simulink library "Linkage_Decoupled_Link5"  (R2025a)
settings: Solver=VariableStepAuto  StartTime=0.0  StopTime=10.0  RelTol=1e-3
undefined symbols (not defined in the file): Init, Left, Linkage, Visual, X, Y, Z
libraries: sm_lib x24, Linkage_Arms x7, Suspension_Utilities x6, Linkage_Uprights x1
(part 1 of 2)
Description:
  | Component of Simscape Vehicle Templates Library
  | 
  | Copyright 2018-2026 The MathWorks, Inc.
settings Model: Creator=smiller  LastModifiedBy=smiller
settings SolverCC: AlgebraicLoopSolver=TrustRegion
settings DataIOCC: ReturnWorkspaceOutputs=off
settings OptimizationCC: ReuseModelBlockBuffer=off
settings DebuggingCC: UnconnectedInputMsg=warning  UnconnectedOutputMsg=warning  UnconnectedLineMsg=warning  ArithmeticOperatorsInVariantConditions=warning
settings ModelReferenceCC: EnableRefExpFcnMdlSchedulingChecks=on
settings SFSimCC: CustomCodeUndefinedFunction=UseInterfaceOnly
settings RTWCC: GPUComputeCapability=3.5

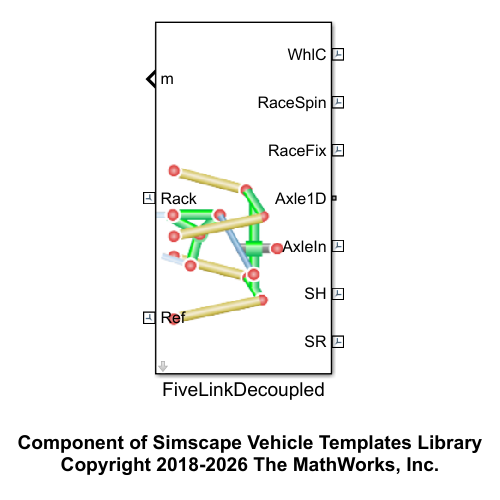
[thumbnail: Simulink's stored preview of the top-level diagram]
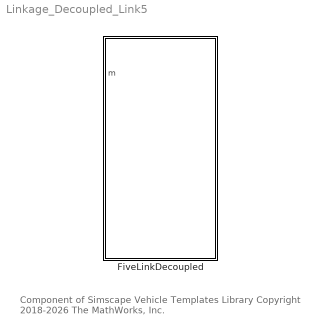
== system Linkage_Decoupled_Link5 ==
  note: Component of Simscape Vehicle Templates Library
      | Copyright 2018-2026 The MathWorks, Inc.
  FiveLinkDecoupled : Subsystem  VariantControl=FiveLinkShockFront  mask(Five-Link Suspension, Decoupled){popup_leftRight=Left, hp_in_f_ua=Linkage.UpperArmF.sInboard.Value, hp_in_r_ua=Linkage.UpperArmR.sInboard.Value, hp_out_f_ua=Linkage.UpperArmF.sOutboard.Value, hp_out_r_ua=Linkage.UpperArmR.sOutboard.Value, hp_in_f_la=Linkage.LowerArmF.sInboard.Value, hp_in_r_la=Linkage.LowerArmR.sInboard.Value, hp_out_f_la=Linkage.LowerArmF.sOutboard.Value, hp_out_r_la=Linkage.LowerArmR.sOutboard.Value, hp_pushrod_in=Linkage.Pushrod.sBellcrank.Value, hp_pushrod_out=Linkage.Pushrod.sUpright.Value, hp_bcr_pivot=Linkage.Bellcrank.sPivot.Value, hp_bcr_shock_heaveL=Linkage.Shock.sHeaveL.Value, hp_bcr_shock_heaveR=Linkage.Shock.sHeaveR.Value, hp_bcr_shock_rollL=Linkage.Shock.sRollL.Value, hp_bcr_shock_rollR=Linkage.Shock.sRollR.Value, hp_upr_cg=Linkage.Upright.sCG.Value, hp_upr_wc=Linkage.Upright.sWheelCentre.Value, hp_in_rod=Linkage.TrackRod.sInboard.Value, hp_upr_rod=Linkage.TrackRod.sOutboard.Value, clr_hp=Visual.hp.clr, opc_hp=Visual.hp.opc, size_hp=Visual.hp.rad, UpperArmF_to_Subframe=Linkage.UpperArmF_to_Subframe, UpperArmR_to_Subframe=Linkage.UpperArmR_to_Subframe, LowerArmF_to_Subframe=Linkage.LowerArmF_to_Subframe, LowerArmR_to_Subframe=Linkage.LowerArmR_to_Subframe, uaf_mass=Linkage.UpperArmF.m.Value, uar_mass=Linkage.UpperArmR.m.Value, laf_mass=Linkage.LowerArmF.m.Value, lar_mass=Linkage.LowerArmR.m.Value, clr_conn_links=Visual.hp.clr, opc_conn_links=Visual.hp.opc, size_conn_links=Visual.hp.rad, clr_uaf=Visual.UpperArm.clr, opc_uaf=Visual.part.opc, radius_uaf=Visual.UpperArm.rad, clr_uar=Visual.UpperArm.clr, opc_uar=Visual.part.opc, radius_uar=Visual.UpperArm.rad, clr_laf=Visual.LowerArm.clr, opc_laf=Visual.part.opc, radius_laf=Visual.LowerArm.rad, clr_lar=Visual.LowerArm.clr, opc_lar=Visual.part.opc, radius_lar=Visual.LowerArm.rad, atoe=Linkage.Upright.aToe.Value, acamber=Linkage.Upright.aCamber.Value, upr_mass=Linkage.Upright.m.Value, axle_len=Linkage.Upright.xAxle.Value, axle_whlc_to_bearing=Linkage.Upright.xWCtoBearing.Value, axle_mass=Linkage.Upright.mAxle.Value, clr_conn_upr=Visual.hp.clr, opc_conn_upr=Visual.hp.opc, size_conn_upr=Visual.hp.rad, clr_upr=Visual.Upright.clr, opc_upr=Visual.part.opc, radius_upr=Visual.Upright.rad, clr_axle=Visual.Axle.clr, opc_axle=Visual.part.opc, radius_axle=Visual.Axle.rad, rod_mass=Linkage.TrackRod.m.Value, clr_conn_rod=Visual.hp.clr, opc_conn_rod=Visual.hp.opc, size_conn_rod=Visual.hp.rad, clr_rod=Visual.TrackRod.clr, opc_rod=Visual.part.opc, radius_rod=Visual.TrackRod.rad, bcr_mass=Linkage.Bellcrank.m.Value, clr_bcr=Visual.Bellcrank.clr, opc_bcr=Visual.part.opc, radius_bcr=Visual.Bellcrank.rad, pushrod_mass=Linkage.Pushrod.m.Value, clr_conn_pushrod=Visual.hp.clr, opc_conn_pushrod=Visual.hp.opc, size_conn_pushrod=Visual.hp.rad, clr_pushrod=Visual.Pushrod.clr, opc_pushrod=Visual.part.opc, radius_pushrod=Visual.Pushrod.rad, whl_init_spd_lr=Init.nWheel.Value}
      mask prompts: popup_leftRight "Left/Right"; hp_in_f_ua "Upper Arm Front [xyz] (m)"; hp_in_r_ua "Upper Arm Rear [xyz] (m)"; hp_out_f_ua "Upper Arm Front Outboard [xyz] (m)"; hp_out_r_ua "Upper Arm Rear Outboard [xyz] (m)"; hp_in_f_la "Lower Arm Front [xyz] (m)"; hp_in_r_la "Lower Arm Rear [xyz] (m)"; hp_out_f_la "Lower Arm Front Outboard [xyz] (m)"; hp_out_r_la "Lower Arm Rear Outboard [xyz] (m)"; hp_pushrod_in "Pushrod Bellcrank [xyz] (m)"; hp_pushrod_out "Pushrod Upright [xyz] (m)"; hp_bcr_pivot "Bellcrank Pivot [xyz] (m)"; hp_bcr_shock_heaveL "Bellcrank Shock Heave Left [xyz] (m)"; hp_bcr_shock_heaveR "Bellcrank Shock Heave Right [xyz] (m)"; hp_bcr_shock_rollL "Bellcrank Shock Roll Left [xyz] (m)"; hp_bcr_shock_rollR "Bellcrank Shock Roll Right [xyz] (m)"; hp_upr_cg "Upright CG [xyz] (m)"; hp_upr_wc "Wheel Center [xyz] (m)"; hp_in_rod "Track Rod Inboard [xyz] (m)"; hp_upr_rod "Track Rod Outboard [xyz] (m)"; atoe "Toe Angle (deg)"; acamber "Camber Angle (deg)"; upr_mass "Mass (kg)"; axle_len "Axle Length (m)"; axle_whlc_to_bearing "Distance Wheel Ctr to Bearing (m)"; axle_mass "Axle Mass (kg)"; rod_mass "Mass (kg)"; bcr_mass "Mass (kg)"; pushrod_mass "Mass (kg)"; whl_init_spd_lr "Initial Wheel Speed (rad/s)"
      mask help: Models a multi-link, decoupled suspension with two upper and two lower control arms connecting the subframe to the upright. Mechanical connections via a bellcrank permit this design to decouple stiffness and damping for body roll and heave.
      mask init:
      | if(popup_leftRight == 1)
      |     rhs_susp = 1;
      |     %whlind = 1;
      |     whl_init_spd = whl_init_spd_lr(1);
      |     hp_bcr_shock_heave = hp_bcr_shock_heaveL;
      |     hp_bcr_shock_roll = hp_bcr_shock_rollL;
      | elseif(popup_leftRight == 2)
      |     rhs_susp = -1;
      |     %whlind = 2;
      | 	whl_init_spd = whl_init_spd_lr(2);
      |     hp_bcr_shock_heave = hp_bcr_shock_heaveR;
      |     hp_bcr_shock_roll = hp_bcr_shock_rollR;    
      | end
      mask TypeOptions popup_leftRight:
      | Hardpoints/popup_leftRight | Upright/popup_leftRight | Lower Arm Rear/popup_leftRight | Lower Arm Front/popup_leftRight | Track Rod/popup_leftRight | Upper Arm Front/popup_leftRight | Upper Arm Rear/popup_leftRight | Universal
      | HP LAF/popup_leftRight | Universal
      | HP LAR/popup_leftRight | Universal
      | HP UAF/popup_leftRight | Universal
      | HP UAR/popup_leftRight | Pushrod/popup_leftRight | Bellcrank/popup_leftRight | HP Bellcrank/popup_leftRight
      mask TypeOptions hp_in_f_ua:
      | Hardpoints/hp_in_f_ua | Universal
      | HP UAF/hp_joint | Upper Arm Front/hp_in
      mask TypeOptions hp_in_r_ua:
      | Hardpoints/hp_in_r_ua | Universal
      | HP UAR/hp_joint | Upper Arm Rear/hp_in
      mask TypeOptions hp_out_f_ua: Upper Arm Front/hp_out | Upright/hp_uaf_out
      mask TypeOptions hp_out_r_ua: Upper Arm Rear/hp_out | Upright/hp_uar_out
      mask TypeOptions hp_in_f_la:
      | Hardpoints/hp_in_f_la | Lower Arm Front/hp_in | Universal
      | HP LAF/hp_joint
      mask TypeOptions hp_in_r_la:
      | Hardpoints/hp_in_r_la | Lower Arm Rear/hp_in | Universal
      | HP LAR/hp_joint
      mask TypeOptions hp_out_f_la: Upright/hp_laf_out | Lower Arm Front/hp_out
      mask TypeOptions hp_out_r_la: Upright/hp_lar_out | Lower Arm Rear/hp_out
      mask TypeOptions hp_pushrod_in: Pushrod/hp_in | Bellcrank/hp_pushrod | HP Bellcrank/hp_pushrod_in
      mask TypeOptions hp_pushrod_out: Pushrod/hp_out | Upright/hp_pushrod
      mask TypeOptions hp_bcr_pivot: Bellcrank/hp_bcr_pivot | HP Bellcrank/hp_bcr_pivot | Hardpoints/hp_bellcrank
      mask TypeOptions hp_upr_cg: Upright/hp_upr_cg
      mask TypeOptions hp_upr_wc: Upright/hp_upr_wc
      mask TypeOptions hp_in_rod: Track Rod/hp_in
      mask TypeOptions hp_upr_rod: Track Rod/hp_out | Upright/hp_upr_rod
      mask TypeOptions clr_hp: Hardpoints/clr_hp
      mask TypeOptions opc_hp: Hardpoints/opc_hp
      mask TypeOptions size_hp: Hardpoints/size_hp
      mask TypeOptions uaf_mass: Upper Arm Front/rod_mass
      mask TypeOptions uar_mass: Upper Arm Rear/rod_mass
      mask TypeOptions laf_mass: Lower Arm Front/rod_mass
      mask TypeOptions lar_mass: Lower Arm Rear/rod_mass
      mask TypeOptions clr_conn_links: Upper Arm Front/clr_conn_rod | Upper Arm Rear/clr_conn_rod | Lower Arm Front/clr_conn_rod | Lower Arm Rear/clr_conn_rod
      mask TypeOptions opc_conn_links: Upper Arm Front/opc_conn_rod | Upper Arm Rear/opc_conn_rod | Lower Arm Front/opc_conn_rod | Lower Arm Rear/opc_conn_rod
      mask TypeOptions size_conn_links: Upper Arm Front/size_conn_rod | Upper Arm Rear/size_conn_rod | Lower Arm Front/size_conn_rod | Lower Arm Rear/size_conn_rod
      mask TypeOptions clr_uaf: Upper Arm Front/clr_rod
      mask TypeOptions opc_uaf: Upper Arm Front/opc_rod
      mask TypeOptions radius_uaf: Upper Arm Front/radius_rod
      mask TypeOptions clr_uar: Upper Arm Rear/clr_rod
      mask TypeOptions opc_uar: Upper Arm Rear/opc_rod
      mask TypeOptions radius_uar: Upper Arm Rear/radius_rod
      mask TypeOptions clr_laf: Lower Arm Front/clr_rod
      mask TypeOptions opc_laf: Lower Arm Front/opc_rod
      mask TypeOptions radius_laf: Lower Arm Front/radius_rod
      mask TypeOptions clr_lar: Lower Arm Rear/clr_rod
      mask TypeOptions opc_lar: Lower Arm Rear/opc_rod
      mask TypeOptions radius_lar: Lower Arm Rear/radius_rod
      mask TypeOptions atoe: Upright/atoe
      mask TypeOptions acamber: Upright/acamber
      mask TypeOptions upr_mass: Upright/upr_mass
      mask TypeOptions axle_len: Upright/axle_len
      mask TypeOptions axle_whlc_to_bearing: Upright/axle_whlc_to_bearing
      mask TypeOptions axle_mass: Upright/axle_mass
      mask TypeOptions clr_conn_upr: Upright/clr_conn_upr
      mask TypeOptions opc_conn_upr: Upright/opc_conn_upr
      mask TypeOptions size_conn_upr: Upright/size_conn_upr
      mask TypeOptions clr_upr: Upright/clr_upr
      mask TypeOptions opc_upr: Upright/opc_upr
      mask TypeOptions radius_upr: Upright/radius_upr
      mask TypeOptions clr_axle: Upright/clr_axle
      mask TypeOptions opc_axle: Upright/opc_axle
      mask TypeOptions radius_axle: Upright/radius_axle
      mask TypeOptions rod_mass: Track Rod/rod_mass
      mask TypeOptions clr_conn_rod: Track Rod/clr_conn_rod
      mask TypeOptions opc_conn_rod: Track Rod/opc_conn_rod
      mask TypeOptions size_conn_rod: Track Rod/size_conn_rod
      mask TypeOptions clr_rod: Track Rod/clr_rod
      mask TypeOptions opc_rod: Track Rod/opc_rod
      mask TypeOptions radius_rod: Track Rod/radius_rod
      mask TypeOptions bcr_mass: Bellcrank/bcr_mass
      mask TypeOptions clr_bcr: Bellcrank/clr_bcr
      mask TypeOptions opc_bcr: Bellcrank/opc_bcr
      mask TypeOptions radius_bcr: Bellcrank/radius_bcr
      mask TypeOptions pushrod_mass: Pushrod/rod_mass
      mask TypeOptions clr_conn_pushrod: Pushrod/clr_conn_rod
      mask TypeOptions opc_conn_pushrod: Pushrod/opc_conn_rod
      mask TypeOptions size_conn_pushrod: Pushrod/size_conn_rod
      mask TypeOptions clr_pushrod: Pushrod/clr_rod
      mask TypeOptions opc_pushrod: Pushrod/opc_rod
      mask TypeOptions radius_pushrod: Pushrod/radius_rod
      mask DialogControl cont_hp Prompt: Hardpoints
      mask DialogControl cont_vis_hp Prompt: Visualization
      mask DialogControl text_clr_hp Prompt: Color [RGB]
      mask DialogControl text_opc_hp Prompt: Opac. (0-1)
      mask DialogControl text_size_hp Prompt: Size (m)
      mask DialogControl text_hp Prompt: Hardpoints
      mask DialogControl cont_links Prompt: Links
      mask DialogControl text_links_part_subf Prompt: Part
      mask DialogControl text_links_subf Prompt: Subframe Connection
      mask DialogControl text_upper_f_subf Prompt: Upper, Front
      mask DialogControl text_upper_r_subf Prompt: Upper, Rear
      mask DialogControl text_lower_f_subf Prompt: Lower, Front
      mask DialogControl text_lower_r_subf Prompt: Lower, Rear
      mask DialogControl text_links_part Prompt: Part
      mask DialogControl text_links_mass Prompt: Mass (kg)
      mask DialogControl text_upper_f Prompt: Upper, Front
      mask DialogControl text_upper_r Prompt: Upper, Rear
      mask DialogControl text_lower_f Prompt: Lower, Front
      mask DialogControl text_lower_r Prompt: Lower, Rear
      mask DialogControl cont_vis_links Prompt: Visualization
      mask DialogControl text_vis_links_clr Prompt: Color [RGB]
      mask DialogControl text_vis_links_opc Prompt: Opacity (0-1)
      mask DialogControl text_vis_links_rad Prompt: Radius (m)
      mask DialogControl text_vis_links_conn Prompt: Connections
      mask DialogControl text_vis_links_uaf Prompt: Upper, Front
      mask DialogControl text_vis_links_uar Prompt: Upper, Rear
      mask DialogControl text_vis_links_laf Prompt: Lower, Front
      mask DialogControl text_vis_links_lar Prompt: Lower, Rear
      mask DialogControl cont_upright Prompt: Upright
      mask DialogControl grp_upright Prompt: Upright
      mask DialogControl grp_upright_axle Prompt: Axle
      mask DialogControl cont_vis_upr Prompt: Visualization
      mask DialogControl text_clr_upr Prompt: Color [RGB]
      mask DialogControl text_opc_upr Prompt: Opac. (0-1)
      mask DialogControl text_size_upr Prompt: Size (m)
      mask DialogControl text_conn_upr Prompt: Connections
      mask DialogControl text_upright Prompt: Upright
      mask DialogControl text_axle Prompt: Axle
      mask DialogControl cont_steer Prompt: Steer
      mask DialogControl grp_rod Prompt: Rod
      mask DialogControl cont_vis_rod Prompt: Visualization
      mask DialogControl text_clr_rod Prompt: Color [RGB]
      mask DialogControl text_opc_rod Prompt: Opac. (0-1)
      mask DialogControl text_size_rod Prompt: Size (m)
      mask DialogControl text_conn_rod Prompt: Connections
      mask DialogControl text_rod_rod Prompt: Rod
      mask DialogControl cont_bellcrank Prompt: Bellcrank
      mask DialogControl grp_bellcrank Prompt: Bellcrank
      mask DialogControl cont_vis_bellcrank Prompt: Visualization
      mask DialogControl text_clr_bellcrank Prompt: Color [RGB]
      mask DialogControl text_opc_bellcrank Prompt: Opac. (0-1)
      mask DialogControl text_size_bellcrank Prompt: Size (m)
      mask DialogControl text_bellcrank Prompt: Bellcrank
      mask DialogControl cont_push Prompt: Pushrod
      mask DialogControl grp_pushrod Prompt: Pushrod
      mask DialogControl cont_vis_pushrod Prompt: Visualization
      mask DialogControl text_clr_pushrod Prompt: Color [RGB]
      mask DialogControl text_opc_pushrod Prompt: Opac. (0-1)
      mask DialogControl text_size_pushrod Prompt: Size (m)
      mask DialogControl text_conn_pushrod Prompt: Connections
      mask DialogControl text_pushrod Prompt: Pushrod
      mask DialogControl cont_initial Prompt: Initial
      mask Display: image('sm_car_vehicle_linkage_5ldec_IMAGE.png');

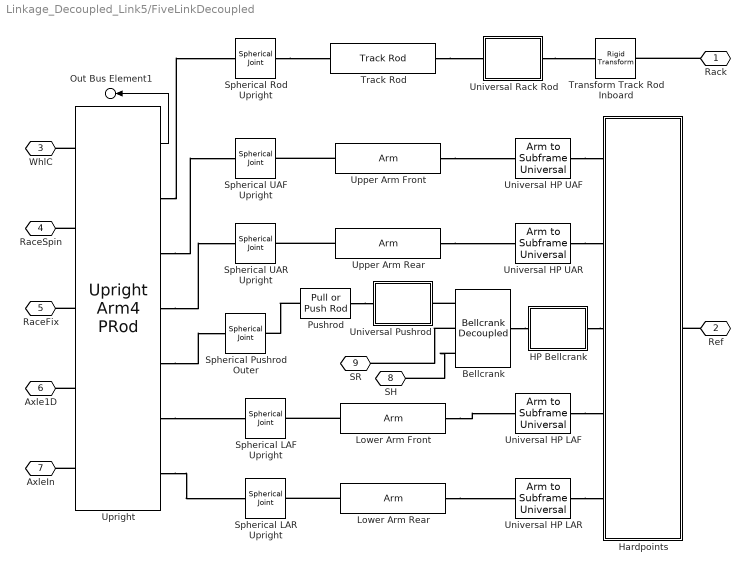
== system Linkage_Decoupled_Link5/FiveLinkDecoupled ==
  Bellcrank : Linkage_Arms/Bellcrank Decoupled  popup_leftRight=Left  hp_bcr_pivot=hp_bcr_pivot  hp_bcr_shock_heave=hp_bcr_shock_heave  hp_bcr_shock_roll=hp_bcr_shock_roll  hp_pushrod=hp_pushrod_in  bcr_mass=bcr_mass  clr_bcr=clr_bcr  opc_bcr=opc_bcr  radius_bcr=radius_bcr
  HP Bellcrank : Subsystem  mask(Revolute Joint 3 Points){popup_leftRight=Left, hp_bcr_pivot=hp_bcr_pivot, hp_pushrod_in=hp_pushrod_in, hp_bcr_shock=hp_bcr_shock_heave}
      mask prompts: popup_leftRight "Left/Right"; hp_bcr_pivot "HP Bellcrank Pivot [xyz] (m)"; hp_pushrod_in "HP Pushrod Inner [xyz] (m)"; hp_bcr_shock "HP Bellcrank Shock Heave [xyz] (m)"
      mask help: Revolute Joint with degree of freedom normal to 3 hardpoints.
      mask init:
      | % Set parameter for mirroring (+y or -y)
      | if(popup_leftRight == 1)
      |     rhs_susp = 1;    
      | elseif(popup_leftRight == 2)
      |     rhs_susp = -1;
      | end
      | 
      | rhs_hp = [1 rhs_susp 1];
      mask TypeOptions popup_leftRight: Left | Right
      mask Display: image('sm_car_variant_revolute.png')
  Hardpoints : Subsystem  mask{popup_leftRight=Left, hp_in_f_ua=hp_in_f_ua, hp_in_r_ua=hp_in_r_ua, hp_in_f_la=hp_in_f_la, hp_in_r_la=hp_in_r_la, hp_bellcrank=hp_bcr_pivot, clr_hp=clr_hp, opc_hp=opc_hp, size_hp=size_hp}
      mask prompts: popup_leftRight "Left/Right"; hp_in_f_ua "Upper Arm Front [xyz] (m)"; hp_in_r_ua "Upper Arm Rear [xyz] (m)"; hp_in_f_la "Lower Arm Front [xyz] (m)"; hp_in_r_la "Lower Arm Rear [xyz] (m)"; hp_bellcrank "Bellcrank Pivot [xyz] (m)"
      mask init:
      | % Set parameter for mirroring (+y or -y)
      | if(popup_leftRight == 1)
      |     rhs_susp = 1;    
      | elseif(popup_leftRight == 2)
      |     rhs_susp = -1;
      | end
      | 
      | rhs_hp = [1 rhs_susp 1];
      mask TypeOptions popup_leftRight: Left | Right
      mask TypeOptions clr_hp: Vis HP LAr/GraphicDiffuseColor | Vis HP Bellcrank/GraphicDiffuseColor | Vis HP UAf/GraphicDiffuseColor | Vis HP UAr/GraphicDiffuseColor | Vis HP LAf/GraphicDiffuseColor
      mask TypeOptions opc_hp: Vis HP LAr/GraphicOpacity | Vis HP Bellcrank/GraphicOpacity | Vis HP UAf/GraphicOpacity | Vis HP UAr/GraphicOpacity | Vis HP LAf/GraphicOpacity
      mask DialogControl cont_hp Prompt: Hardpoints
      mask DialogControl cont_vis_hp Prompt: Visualization
      mask DialogControl text_clr_hp Prompt: Color [RGB]
      mask DialogControl text_opc_hp Prompt: Opac. (0-1)
      mask DialogControl text_size_hp Prompt: Size (m)
      mask DialogControl text_hp Prompt: Hardpoints
      mask Display: image('sm_car_vehicle_linkage_link5_hp_IMAGE.png');
  Lower Arm Front : Linkage_Arms/Arm  VariantControl=Steer  popup_leftRight=Left  hp_in=hp_in_f_la  hp_out=hp_out_f_la  rod_mass=laf_mass  clr_conn_rod=clr_conn_links  opc_conn_rod=opc_conn_links  size_conn_rod=size_conn_links  clr_rod=clr_laf  opc_rod=opc_laf  radius_rod=radius_laf
  Lower Arm Rear : Linkage_Arms/Arm  VariantControl=Steer  popup_leftRight=Left  hp_in=hp_in_r_la  hp_out=hp_out_r_la  rod_mass=lar_mass  clr_conn_rod=clr_conn_links  opc_conn_rod=opc_conn_links  size_conn_rod=size_conn_links  clr_rod=clr_lar  opc_rod=opc_lar  radius_rod=radius_lar
  Pushrod : Linkage_Arms/Pull or Push Rod  VariantControl=Steer  popup_leftRight=Left  hp_in=hp_pushrod_in  hp_out=hp_pushrod_out  rod_mass=pushrod_mass  clr_conn_rod=clr_conn_pushrod  opc_conn_rod=opc_conn_pushrod  size_conn_rod=size_conn_pushrod  clr_rod=clr_pushrod  opc_rod=opc_pushrod  radius_rod=radius_pushrod
  Spherical LAF Upright : sm_lib/Joints/Spherical Joint  JointMode=Normal  CompositeWrenchDir=FollowerOnBase  CompositeWrenchFrame=BaseFrame  SenseConstraintForce=off  SenseConstraintTorque=off  SenseTotalForce=off  SenseTotalTorque=off  PositionTargetSpecify=on  PositionTargetPriority=Low  PositionTargetRotationMethod=None  PositionTargetFollAlignAxisA=+X  PositionTargetBaseAlignAxisA=+Y  PositionTargetFollAlignAxisB=+Y  PositionTargetBaseAlignAxisB=+Z  PositionTargetRotationStandardAxis=+Z  PositionTargetRotationAngle=0.0  PositionTargetRotationAngleUnits=deg  PositionTargetRotationArbitraryAxis=[0 0 1]  PositionTargetRotationSequenceAxes=FollowerAxes  PositionTargetRotationSequence=XYX  PositionTargetRotationSequenceAngles=[0 0 0]  PositionTargetRotationSequenceAnglesUnits=deg  PositionTargetRotationMatrix=[1 0 0; 0 1 0; 0 0 1]  PositionTargetQuaternion=[1 0 0 0]  VelocityTargetSpecify=off  VelocityTargetPriority=High  VelocityTargetValue=[0 0 0]  VelocityTargetValueUnits=deg/s  VelocityTargetInFollowerFrame=on  EqPosRotationMethod=None  EqPosFollAlignAxisA=+X  EqPosBaseAlignAxisA=+Y  EqPosFollAlignAxisB=+Y  EqPosBaseAlignAxisB=+Z  EqPosRotationStandardAxis=+Z  EqPosRotationAngle=0.0  EqPosRotationAngleUnits=deg  EqPosRotationArbitraryAxis=[0 0 1]  EqPosRotationSequenceAxes=FollowerAxes  EqPosRotationSequence=XYX  EqPosRotationSequenceAngles=[0 0 0]  EqPosRotationSequenceAnglesUnits=deg  EqPosRotationMatrix=[1 0 0; 0 1 0; 0 0 1]  EqPosQuaternion=[1 0 0 0]  SpringStiffness=0  SpringStiffnessUnits=N*m/deg  DampingCoefficient=0  DampingCoefficientUnits=N*m/(deg/s)  LowerLimitSpecify=off  LowerLimitBound=15  LowerLimitBoundUnits=deg  LowerLimitStiffness=1e4  LowerLimitStiffnessUnits=N*m/deg  LowerLimitDamping=10  LowerLimitDampingUnits=N*m/(deg/s)  LowerLimitTransitionRegionWidth=0.1  LowerLimitTransitionRegionWidthUnits=deg  UpperLimitSpecify=off  UpperLimitBound=45  UpperLimitBoundUnits=deg  UpperLimitStiffness=1e4  UpperLimitStiffnessUnits=N*m/deg  UpperLimitDamping=10  UpperLimitDampingUnits=N*m/(deg/s)  UpperLimitTransitionRegionWidth=0.1  UpperLimitTransitionRegionWidthUnits=deg  TorqueActuationMode=NoTorque  ActuateTorqueX=off  ActuateTorqueY=off  ActuateTorqueZ=off  ActuateTorque=off  ActuationFrame=BaseFrame  SensePosition=off  SenseVelocityX=off  SenseVelocityY=off  SenseVelocityZ=off  SenseVelocity=off  SenseAccelerationX=off  SenseAccelerationY=off  SenseAccelerationZ=off  SenseAcceleration=off  SenseLowerLimitTorqueMag=off  SenseUpperLimitTorqueMag=off  SensingFrame=BaseFrame
  Spherical LAR Upright : sm_lib/Joints/Spherical Joint  JointMode=Normal  CompositeWrenchDir=FollowerOnBase  CompositeWrenchFrame=BaseFrame  SenseConstraintForce=off  SenseConstraintTorque=off  SenseTotalForce=off  SenseTotalTorque=off  PositionTargetSpecify=on  PositionTargetPriority=Low  PositionTargetRotationMethod=None  PositionTargetFollAlignAxisA=+X  PositionTargetBaseAlignAxisA=+Y  PositionTargetFollAlignAxisB=+Y  PositionTargetBaseAlignAxisB=+Z  PositionTargetRotationStandardAxis=+Z  PositionTargetRotationAngle=0.0  PositionTargetRotationAngleUnits=deg  PositionTargetRotationArbitraryAxis=[0 0 1]  PositionTargetRotationSequenceAxes=FollowerAxes  PositionTargetRotationSequence=XYX  PositionTargetRotationSequenceAngles=[0 0 0]  PositionTargetRotationSequenceAnglesUnits=deg  PositionTargetRotationMatrix=[1 0 0; 0 1 0; 0 0 1]  PositionTargetQuaternion=[1 0 0 0]  VelocityTargetSpecify=off  VelocityTargetPriority=High  VelocityTargetValue=[0 0 0]  VelocityTargetValueUnits=deg/s  VelocityTargetInFollowerFrame=on  EqPosRotationMethod=None  EqPosFollAlignAxisA=+X  EqPosBaseAlignAxisA=+Y  EqPosFollAlignAxisB=+Y  EqPosBaseAlignAxisB=+Z  EqPosRotationStandardAxis=+Z  EqPosRotationAngle=0.0  EqPosRotationAngleUnits=deg  EqPosRotationArbitraryAxis=[0 0 1]  EqPosRotationSequenceAxes=FollowerAxes  EqPosRotationSequence=XYX  EqPosRotationSequenceAngles=[0 0 0]  EqPosRotationSequenceAnglesUnits=deg  EqPosRotationMatrix=[1 0 0; 0 1 0; 0 0 1]  EqPosQuaternion=[1 0 0 0]  SpringStiffness=0  SpringStiffnessUnits=N*m/deg  DampingCoefficient=0  DampingCoefficientUnits=N*m/(deg/s)  LowerLimitSpecify=off  LowerLimitBound=15  LowerLimitBoundUnits=deg  LowerLimitStiffness=1e4  LowerLimitStiffnessUnits=N*m/deg  LowerLimitDamping=10  LowerLimitDampingUnits=N*m/(deg/s)  LowerLimitTransitionRegionWidth=0.1  LowerLimitTransitionRegionWidthUnits=deg  UpperLimitSpecify=off  UpperLimitBound=45  UpperLimitBoundUnits=deg  UpperLimitStiffness=1e4  UpperLimitStiffnessUnits=N*m/deg  UpperLimitDamping=10  UpperLimitDampingUnits=N*m/(deg/s)  UpperLimitTransitionRegionWidth=0.1  UpperLimitTransitionRegionWidthUnits=deg  TorqueActuationMode=NoTorque  ActuateTorqueX=off  ActuateTorqueY=off  ActuateTorqueZ=off  ActuateTorque=off  ActuationFrame=BaseFrame  SensePosition=off  SenseVelocityX=off  SenseVelocityY=off  SenseVelocityZ=off  SenseVelocity=off  SenseAccelerationX=off  SenseAccelerationY=off  SenseAccelerationZ=off  SenseAcceleration=off  SenseLowerLimitTorqueMag=off  SenseUpperLimitTorqueMag=off  SensingFrame=BaseFrame
  Spherical Pushrod Outer : sm_lib/Joints/Spherical Joint  JointMode=Normal  CompositeWrenchDir=FollowerOnBase  CompositeWrenchFrame=BaseFrame  SenseConstraintForce=off  SenseConstraintTorque=off  SenseTotalForce=off  SenseTotalTorque=off  PositionTargetSpecify=on  PositionTargetPriority=Low  PositionTargetRotationMethod=AlignedAxes  PositionTargetFollAlignAxisA=+X  PositionTargetBaseAlignAxisA=+X  PositionTargetFollAlignAxisB=+Y  PositionTargetBaseAlignAxisB=+Y  PositionTargetRotationStandardAxis=+Z  PositionTargetRotationAngle=0.0  PositionTargetRotationAngleUnits=deg  PositionTargetRotationArbitraryAxis=[0 0 1]  PositionTargetRotationSequenceAxes=FollowerAxes  PositionTargetRotationSequence=XYX  PositionTargetRotationSequenceAngles=[0 0 0]  PositionTargetRotationSequenceAnglesUnits=deg  PositionTargetRotationMatrix=[1 0 0; 0 1 0; 0 0 1]  PositionTargetQuaternion=[1 0 0 0]  VelocityTargetSpecify=off  VelocityTargetPriority=High  VelocityTargetValue=[0 0 0]  VelocityTargetValueUnits=deg/s  VelocityTargetInFollowerFrame=on  EqPosRotationMethod=None  EqPosFollAlignAxisA=+X  EqPosBaseAlignAxisA=+Y  EqPosFollAlignAxisB=+Y  EqPosBaseAlignAxisB=+Z  EqPosRotationStandardAxis=+Z  EqPosRotationAngle=0.0  EqPosRotationAngleUnits=deg  EqPosRotationArbitraryAxis=[0 0 1]  EqPosRotationSequenceAxes=FollowerAxes  EqPosRotationSequence=XYX  EqPosRotationSequenceAngles=[0 0 0]  EqPosRotationSequenceAnglesUnits=deg  EqPosRotationMatrix=[1 0 0; 0 1 0; 0 0 1]  EqPosQuaternion=[1 0 0 0]  SpringStiffness=0  SpringStiffnessUnits=N*m/deg  DampingCoefficient=0  DampingCoefficientUnits=N*m/(deg/s)  LowerLimitSpecify=off  LowerLimitBound=15  LowerLimitBoundUnits=deg  LowerLimitStiffness=1e4  LowerLimitStiffnessUnits=N*m/deg  LowerLimitDamping=10  LowerLimitDampingUnits=N*m/(deg/s)  LowerLimitTransitionRegionWidth=0.1  LowerLimitTransitionRegionWidthUnits=deg  UpperLimitSpecify=off  UpperLimitBound=45  UpperLimitBoundUnits=deg  UpperLimitStiffness=1e4  UpperLimitStiffnessUnits=N*m/deg  UpperLimitDamping=10  UpperLimitDampingUnits=N*m/(deg/s)  UpperLimitTransitionRegionWidth=0.1  UpperLimitTransitionRegionWidthUnits=deg  TorqueActuationMode=NoTorque  ActuateTorqueX=off  ActuateTorqueY=off  ActuateTorqueZ=off  ActuateTorque=off  ActuationFrame=BaseFrame  SensePosition=off  SenseVelocityX=off  SenseVelocityY=off  SenseVelocityZ=off  SenseVelocity=off  SenseAccelerationX=off  SenseAccelerationY=off  SenseAccelerationZ=off  SenseAcceleration=off  SenseLowerLimitTorqueMag=off  SenseUpperLimitTorqueMag=off  SensingFrame=BaseFrame
  Spherical Rod Upright : sm_lib/Joints/Spherical Joint  JointMode=Normal  CompositeWrenchDir=FollowerOnBase  CompositeWrenchFrame=BaseFrame  SenseConstraintForce=off  SenseConstraintTorque=off  SenseTotalForce=off  SenseTotalTorque=off  PositionTargetSpecify=off  PositionTargetPriority=High  PositionTargetRotationMethod=None  PositionTargetFollAlignAxisA=+X  PositionTargetBaseAlignAxisA=+Y  PositionTargetFollAlignAxisB=+Y  PositionTargetBaseAlignAxisB=+Z  PositionTargetRotationStandardAxis=+Z  PositionTargetRotationAngle=0.0  PositionTargetRotationAngleUnits=deg  PositionTargetRotationArbitraryAxis=[0 0 1]  PositionTargetRotationSequenceAxes=FollowerAxes  PositionTargetRotationSequence=XYX  PositionTargetRotationSequenceAngles=[0 0 0]  PositionTargetRotationSequenceAnglesUnits=deg  PositionTargetRotationMatrix=[1 0 0; 0 1 0; 0 0 1]  PositionTargetQuaternion=[1 0 0 0]  VelocityTargetSpecify=off  VelocityTargetPriority=High  VelocityTargetValue=[0 0 0]  VelocityTargetValueUnits=deg/s  VelocityTargetInFollowerFrame=on  EqPosRotationMethod=None  EqPosFollAlignAxisA=+X  EqPosBaseAlignAxisA=+Y  EqPosFollAlignAxisB=+Y  EqPosBaseAlignAxisB=+Z  EqPosRotationStandardAxis=+Z  EqPosRotationAngle=0.0  EqPosRotationAngleUnits=deg  EqPosRotationArbitraryAxis=[0 0 1]  EqPosRotationSequenceAxes=FollowerAxes  EqPosRotationSequence=XYX  EqPosRotationSequenceAngles=[0 0 0]  EqPosRotationSequenceAnglesUnits=deg  EqPosRotationMatrix=[1 0 0; 0 1 0; 0 0 1]  EqPosQuaternion=[1 0 0 0]  SpringStiffness=0  SpringStiffnessUnits=N*m/deg  DampingCoefficient=0  DampingCoefficientUnits=N*m/(deg/s)  LowerLimitSpecify=off  LowerLimitBound=15  LowerLimitBoundUnits=deg  LowerLimitStiffness=1e4  LowerLimitStiffnessUnits=N*m/deg  LowerLimitDamping=10  LowerLimitDampingUnits=N*m/(deg/s)  LowerLimitTransitionRegionWidth=0.1  LowerLimitTransitionRegionWidthUnits=deg  UpperLimitSpecify=off  UpperLimitBound=45  UpperLimitBoundUnits=deg  UpperLimitStiffness=1e4  UpperLimitStiffnessUnits=N*m/deg  UpperLimitDamping=10  UpperLimitDampingUnits=N*m/(deg/s)  UpperLimitTransitionRegionWidth=0.1  UpperLimitTransitionRegionWidthUnits=deg  TorqueActuationMode=NoTorque  ActuateTorqueX=off  ActuateTorqueY=off  ActuateTorqueZ=off  ActuateTorque=off  ActuationFrame=BaseFrame  SensePosition=off  SenseVelocityX=off  SenseVelocityY=off  SenseVelocityZ=off  SenseVelocity=off  SenseAccelerationX=off  SenseAccelerationY=off  SenseAccelerationZ=off  SenseAcceleration=off  SenseLowerLimitTorqueMag=off  SenseUpperLimitTorqueMag=off  SensingFrame=BaseFrame
  Spherical UAF Upright : sm_lib/Joints/Spherical Joint  JointMode=Normal  CompositeWrenchDir=FollowerOnBase  CompositeWrenchFrame=BaseFrame  SenseConstraintForce=off  SenseConstraintTorque=off  SenseTotalForce=off  SenseTotalTorque=off  PositionTargetSpecify=on  PositionTargetPriority=Low  PositionTargetRotationMethod=None  PositionTargetFollAlignAxisA=+X  PositionTargetBaseAlignAxisA=+Y  PositionTargetFollAlignAxisB=+Y  PositionTargetBaseAlignAxisB=+Z  PositionTargetRotationStandardAxis=+Z  PositionTargetRotationAngle=0.0  PositionTargetRotationAngleUnits=deg  PositionTargetRotationArbitraryAxis=[0 0 1]  PositionTargetRotationSequenceAxes=FollowerAxes  PositionTargetRotationSequence=XYX  PositionTargetRotationSequenceAngles=[0 0 0]  PositionTargetRotationSequenceAnglesUnits=deg  PositionTargetRotationMatrix=[1 0 0; 0 1 0; 0 0 1]  PositionTargetQuaternion=[1 0 0 0]  VelocityTargetSpecify=off  VelocityTargetPriority=High  VelocityTargetValue=[0 0 0]  VelocityTargetValueUnits=deg/s  VelocityTargetInFollowerFrame=on  EqPosRotationMethod=None  EqPosFollAlignAxisA=+X  EqPosBaseAlignAxisA=+Y  EqPosFollAlignAxisB=+Y  EqPosBaseAlignAxisB=+Z  EqPosRotationStandardAxis=+Z  EqPosRotationAngle=0.0  EqPosRotationAngleUnits=deg  EqPosRotationArbitraryAxis=[0 0 1]  EqPosRotationSequenceAxes=FollowerAxes  EqPosRotationSequence=XYX  EqPosRotationSequenceAngles=[0 0 0]  EqPosRotationSequenceAnglesUnits=deg  EqPosRotationMatrix=[1 0 0; 0 1 0; 0 0 1]  EqPosQuaternion=[1 0 0 0]  SpringStiffness=0  SpringStiffnessUnits=N*m/deg  DampingCoefficient=0  DampingCoefficientUnits=N*m/(deg/s)  LowerLimitSpecify=off  LowerLimitBound=15  LowerLimitBoundUnits=deg  LowerLimitStiffness=1e4  LowerLimitStiffnessUnits=N*m/deg  LowerLimitDamping=10  LowerLimitDampingUnits=N*m/(deg/s)  LowerLimitTransitionRegionWidth=0.1  LowerLimitTransitionRegionWidthUnits=deg  UpperLimitSpecify=off  UpperLimitBound=45  UpperLimitBoundUnits=deg  UpperLimitStiffness=1e4  UpperLimitStiffnessUnits=N*m/deg  UpperLimitDamping=10  UpperLimitDampingUnits=N*m/(deg/s)  UpperLimitTransitionRegionWidth=0.1  UpperLimitTransitionRegionWidthUnits=deg  TorqueActuationMode=NoTorque  ActuateTorqueX=off  ActuateTorqueY=off  ActuateTorqueZ=off  ActuateTorque=off  ActuationFrame=BaseFrame  SensePosition=off  SenseVelocityX=off  SenseVelocityY=off  SenseVelocityZ=off  SenseVelocity=off  SenseAccelerationX=off  SenseAccelerationY=off  SenseAccelerationZ=off  SenseAcceleration=off  SenseLowerLimitTorqueMag=off  SenseUpperLimitTorqueMag=off  SensingFrame=BaseFrame
  Spherical UAR Upright : sm_lib/Joints/Spherical Joint  JointMode=Normal  CompositeWrenchDir=FollowerOnBase  CompositeWrenchFrame=BaseFrame  SenseConstraintForce=off  SenseConstraintTorque=off  SenseTotalForce=off  SenseTotalTorque=off  PositionTargetSpecify=on  PositionTargetPriority=Low  PositionTargetRotationMethod=None  PositionTargetFollAlignAxisA=+X  PositionTargetBaseAlignAxisA=+X  PositionTargetFollAlignAxisB=+Y  PositionTargetBaseAlignAxisB=+Y  PositionTargetRotationStandardAxis=+Z  PositionTargetRotationAngle=0.0  PositionTargetRotationAngleUnits=deg  PositionTargetRotationArbitraryAxis=[0 0 1]  PositionTargetRotationSequenceAxes=FollowerAxes  PositionTargetRotationSequence=XYX  PositionTargetRotationSequenceAngles=[0 0 0]  PositionTargetRotationSequenceAnglesUnits=deg  PositionTargetRotationMatrix=[1 0 0; 0 1 0; 0 0 1]  PositionTargetQuaternion=[1 0 0 0]  VelocityTargetSpecify=off  VelocityTargetPriority=High  VelocityTargetValue=[0 0 0]  VelocityTargetValueUnits=deg/s  VelocityTargetInFollowerFrame=on  EqPosRotationMethod=None  EqPosFollAlignAxisA=+X  EqPosBaseAlignAxisA=+Y  EqPosFollAlignAxisB=+Y  EqPosBaseAlignAxisB=+Z  EqPosRotationStandardAxis=+Z  EqPosRotationAngle=0.0  EqPosRotationAngleUnits=deg  EqPosRotationArbitraryAxis=[0 0 1]  EqPosRotationSequenceAxes=FollowerAxes  EqPosRotationSequence=XYX  EqPosRotationSequenceAngles=[0 0 0]  EqPosRotationSequenceAnglesUnits=deg  EqPosRotationMatrix=[1 0 0; 0 1 0; 0 0 1]  EqPosQuaternion=[1 0 0 0]  SpringStiffness=0  SpringStiffnessUnits=N*m/deg  DampingCoefficient=0  DampingCoefficientUnits=N*m/(deg/s)  LowerLimitSpecify=off  LowerLimitBound=15  LowerLimitBoundUnits=deg  LowerLimitStiffness=1e4  LowerLimitStiffnessUnits=N*m/deg  LowerLimitDamping=10  LowerLimitDampingUnits=N*m/(deg/s)  LowerLimitTransitionRegionWidth=0.1  LowerLimitTransitionRegionWidthUnits=deg  UpperLimitSpecify=off  UpperLimitBound=45  UpperLimitBoundUnits=deg  UpperLimitStiffness=1e4  UpperLimitStiffnessUnits=N*m/deg  UpperLimitDamping=10  UpperLimitDampingUnits=N*m/(deg/s)  UpperLimitTransitionRegionWidth=0.1  UpperLimitTransitionRegionWidthUnits=deg  TorqueActuationMode=NoTorque  ActuateTorqueX=off  ActuateTorqueY=off  ActuateTorqueZ=off  ActuateTorque=off  ActuationFrame=BaseFrame  SensePosition=off  SenseVelocityX=off  SenseVelocityY=off  SenseVelocityZ=off  SenseVelocity=off  SenseAccelerationX=off  SenseAccelerationY=off  SenseAccelerationZ=off  SenseAcceleration=off  SenseLowerLimitTorqueMag=off  SenseUpperLimitTorqueMag=off  SensingFrame=BaseFrame
  Track Rod : Linkage_Arms/Track Rod  VariantControl=Steer  popup_leftRight=Left  hp_in=hp_in_rod  hp_out=hp_upr_rod  rod_mass=rod_mass  clr_conn_rod=clr_conn_rod  opc_conn_rod=opc_conn_rod  size_conn_rod=size_conn_rod  clr_rod=clr_rod  opc_rod=opc_rod  radius_rod=radius_rod
  Transform Track Rod Inboard : sm_lib/Frames and Transforms/Rigid Transform  RotationMethod=None  FollAlignAxisA=+X  BaseAlignAxisA=+Y  FollAlignAxisB=+Y  BaseAlignAxisB=+Z  RotationStandardAxis=+Z  RotationAngle=0.0  RotationAngleUnits=deg  RotationArbitraryAxis=[0 0 1]  RotationSequenceAxes=FollowerAxes  RotationSequence=XYX  RotationSequenceAngles=[0 0 0]  RotationSequenceAnglesUnits=deg  RotationMatrix=[1 0 0; 0 1 0; 0 0 1]  Quaternion=[1 0 0 0]  TranslationMethod=Cartesian  TranslationCartesianOffset=hp_in_rod.*[1 rhs_susp 1]  TranslationCartesianOffsetUnits=m  TranslationStandardAxis=+Z  TranslationStandardOffset=0  TranslationStandardOffsetUnits=m  TranslationROffset=0  TranslationROffsetUnits=m  TranslationThetaOffset=0  TranslationThetaOffsetUnits=deg  TranslationZOffset=0  TranslationZOffsetUnits=m
  Universal HP LAF : Suspension_Utilities/Arm to Subframe Universal  VariantControl=Variant1  LabelModeActiveChoice=Bushing_AxRad  popup_leftRight=Left  hp_joint=hp_in_f_la  Connection=LowerArmF_to_Subframe  VariantLabel=LowerArmF_to_Subframe.class.Value  checkbox_setTargets=off
      settings: AttributesFormatString=%<ActiveVariant>
  Universal HP LAR : Suspension_Utilities/Arm to Subframe Universal  VariantControl=Variant1  LabelModeActiveChoice=Bushing_AxRad  popup_leftRight=Left  hp_joint=hp_in_r_la  Connection=LowerArmR_to_Subframe  VariantLabel=LowerArmR_to_Subframe.class.Value  checkbox_setTargets=off
      settings: AttributesFormatString=%<ActiveVariant>
  Universal HP UAF : Suspension_Utilities/Arm to Subframe Universal  VariantControl=Variant1  LabelModeActiveChoice=Bushing_AxRad  popup_leftRight=Left  hp_joint=hp_in_f_ua  Connection=UpperArmF_to_Subframe  VariantLabel=UpperArmF_to_Subframe.class.Value  checkbox_setTargets=on
      settings: AttributesFormatString=%<ActiveVariant>
  Universal HP UAR : Suspension_Utilities/Arm to Subframe Universal  VariantControl=Variant1  LabelModeActiveChoice=Bushing_AxRad  popup_leftRight=Left  hp_joint=hp_in_r_ua  Connection=UpperArmR_to_Subframe  VariantLabel=UpperArmR_to_Subframe.class.Value  checkbox_setTargets=off
      settings: AttributesFormatString=%<ActiveVariant>
  Universal Pushrod : Subsystem
      mask Display: image('sm_car_variant_universal.png');
  Universal Rack Rod : Subsystem
      mask Display: image('sm_car_variant_universal.png');
  Upper Arm Front : Linkage_Arms/Arm  VariantControl=Steer  popup_leftRight=Left  hp_in=hp_in_f_ua  hp_out=hp_out_f_ua  rod_mass=uaf_mass  clr_conn_rod=clr_conn_links  opc_conn_rod=opc_conn_links  size_conn_rod=size_conn_links  clr_rod=clr_uaf  opc_rod=opc_uaf  radius_rod=radius_uaf
  Upper Arm Rear : Linkage_Arms/Arm  VariantControl=Steer  popup_leftRight=Left  hp_in=hp_in_r_ua  hp_out=hp_out_r_ua  rod_mass=uar_mass  clr_conn_rod=clr_conn_links  opc_conn_rod=opc_conn_links  size_conn_rod=size_conn_links  clr_rod=clr_uar  opc_rod=opc_uar  radius_rod=radius_uar
  Upright : Linkage_Uprights/Upright Arm4 PRod  popup_leftRight=Left  hp_uaf_out=hp_out_f_ua  hp_uar_out=hp_out_r_ua  hp_laf_out=hp_out_f_la  hp_lar_out=hp_out_r_la  hp_pushrod=hp_pushrod_out  hp_upr_rod=hp_upr_rod  hp_upr_cg=hp_upr_cg  hp_upr_wc=hp_upr_wc  axle_len=axle_len  axle_whlc_to_bearing=axle_whlc_to_bearing  axle_mass=axle_mass  atoe=atoe  acamber=acamber  upr_mass=upr_mass  whl_init_spd_upr=whl_init_spd  clr_conn_upr=clr_conn_upr  opc_conn_upr=opc_conn_upr  size_conn_upr=size_conn_upr  clr_upr=clr_upr  opc_upr=opc_upr  radius_upr=radius_upr  clr_axle=clr_axle  opc_axle=opc_axle  radius_axle=radius_axle
  Rack : PMIOPort  Side=Right
  Ref : PMIOPort  Port=2  Side=Right
  WhlC : PMIOPort  Port=3  Side=Left
  RaceSpin : PMIOPort  Port=4  Side=Left
  RaceFix : PMIOPort  Port=5  Side=Left
  Axle1D : PMIOPort  Port=6  Side=Left
  AxleIn : PMIOPort  Port=7  Side=Left
  SH : PMIOPort  Port=8  Side=Left
  SR : PMIOPort  Port=9  Side=Left
  Out Bus Element1 : Outport  VectorParamsAs1DForOutWhenUnconnected=off  PortName=m  Element=Upright
  wires:
  Upright/1 -> Out Bus Element1/1
  connections:
  Upright/LConn5 -- AxleIn/RConn1
  Upright/LConn3 -- RaceFix/RConn1
  Upright/LConn2 -- RaceSpin/RConn1
  Track Rod/RConn1 -- Universal Rack Rod/LConn1
  Spherical Rod Upright/LConn1 -- Track Rod/LConn1
  Upright/RConn2 -- Spherical UAF Upright/RConn1
  Lower Arm Front/LConn1 -- Spherical LAF Upright/LConn1
  Upright/RConn5 -- Spherical LAF Upright/RConn1
  Lower Arm Front/RConn1 -- Universal HP LAF/RConn1
  Upright/LConn4 -- Axle1D/RConn1
  Rack/RConn1 -- Transform Track Rod Inboard/LConn1
  Upright/RConn1 -- Spherical Rod Upright/RConn1
  Universal HP UAF/LConn1 -- Hardpoints/LConn1
  Ref/RConn1 -- Hardpoints/RConn1
  HP Bellcrank/LConn1 -- Hardpoints/LConn3
  Upright/LConn1 -- WhlC/RConn1
  Upright/RConn6 -- Spherical LAR Upright/RConn1
  Lower Arm Rear/LConn1 -- Spherical LAR Upright/LConn1
  Universal HP LAR/LConn1 -- Hardpoints/LConn5
  Upper Arm Rear/RConn1 -- Universal HP UAR/RConn1
  Upper Arm Front/LConn1 -- Spherical UAF Upright/LConn1
  Upper Arm Rear/LConn1 -- Spherical UAR Upright/LConn1
  Upright/RConn3 -- Spherical UAR Upright/RConn1
  Universal HP UAR/LConn1 -- Hardpoints/LConn2
  Upper Arm Front/RConn1 -- Universal HP UAF/RConn1
  Universal HP LAF/LConn1 -- Hardpoints/LConn4
  Lower Arm Rear/RConn1 -- Universal HP LAR/RConn1
  Universal Rack Rod/RConn1 -- Transform Track Rod Inboard/RConn1
  Pushrod/LConn1 -- Spherical Pushrod Outer/LConn1
  Upright/RConn4 -- Spherical Pushrod Outer/RConn1
  Bellcrank/RConn1 -- HP Bellcrank/RConn1
  Bellcrank/LConn3 -- SH/RConn1
  Bellcrank/LConn1 -- Universal Pushrod/RConn1
  Pushrod/RConn1 -- Universal Pushrod/LConn1
  Bellcrank/LConn2 -- SR/RConn1

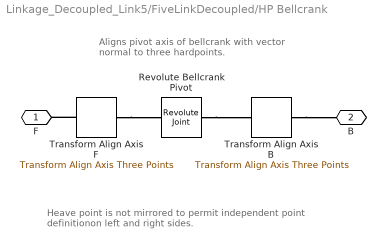
== system Linkage_Decoupled_Link5/FiveLinkDecoupled/HP Bellcrank ==
  note: Heave point is not mirrored to permit independent point definitionon left and right sides.
  note: Aligns pivot axis of bellcrank with vector normal to three hardpoints.
  Revolute Bellcrank Pivot : sm_lib/Joints/Revolute Joint  JointMode=Normal  CompositeWrenchDir=FollowerOnBase  CompositeWrenchFrame=BaseFrame  SenseConstraintForce=off  SenseConstraintTorque=off  SenseTotalForce=off  SenseTotalTorque=off  PositionTargetSpecify=off  PositionTargetPriority=Low  PositionTargetValue=0  PositionTargetValueUnits=deg  VelocityTargetSpecify=off  VelocityTargetPriority=High  VelocityTargetValue=0  VelocityTargetValueUnits=deg/s  EquilibriumPosition=0  EquilibriumPositionUnits=deg  SpringStiffness=0  SpringStiffnessUnits=N*m/deg  DampingCoefficient=0  DampingCoefficientUnits=N*m/(deg/s)  LowerLimitSpecify=off  LowerLimitBound=-90  LowerLimitBoundUnits=deg  LowerLimitStiffness=1e4  LowerLimitStiffnessUnits=N*m/deg  LowerLimitDamping=10  LowerLimitDampingUnits=N*m/(deg/s)  LowerLimitTransitionRegionWidth=0.1  LowerLimitTransitionRegionWidthUnits=deg  UpperLimitSpecify=off  UpperLimitBound=90  UpperLimitBoundUnits=deg  UpperLimitStiffness=1e4  UpperLimitStiffnessUnits=N*m/deg  UpperLimitDamping=10  UpperLimitDampingUnits=N*m/(deg/s)  UpperLimitTransitionRegionWidth=0.1  UpperLimitTransitionRegionWidthUnits=deg  TorqueActuationMode=NoTorque  MotionActuationMode=ComputedMotion  SensePosition=off  SenseVelocity=off  SenseAcceleration=off  SenseTorqueForce=off  SenseLowerLimitTorqueForce=off  SenseUpperLimitTorqueForce=off
  Transform Align Axis B : Suspension_Utilities/Transform Align Axis Three Points  pt1=hp_bcr_pivot.*rhs_hp  pt2=hp_pushrod_in.*rhs_hp  pt3=hp_bcr_shock  popup_f_axis=+Z
  Transform Align Axis F : Suspension_Utilities/Transform Align Axis Three Points  pt1=hp_bcr_pivot.*rhs_hp  pt2=hp_pushrod_in.*rhs_hp  pt3=hp_bcr_shock  popup_f_axis=+Z
  F : PMIOPort  Side=Right
  B : PMIOPort  Port=2  Side=Left
  connections:
  Transform Align Axis F/LConn1 -- F/RConn1
  Revolute Bellcrank Pivot/LConn1 -- Transform Align Axis B/RConn1
  Transform Align Axis F/RConn1 -- Revolute Bellcrank Pivot/RConn1
  Transform Align Axis B/LConn1 -- B/RConn1
